simulink model "untitled_restored_from_autosave"  (R2021b)
settings: Solver=VariableStepAuto  StartTime=0.0  StopTime=100  RelTol=1e-3
libraries: uavalgslib x2, robotcorelib x1, simulink_extras x1, uavutilslib x1
settings Model: Creator=Jihoon Lee  LastModifiedBy=Jihoon Lee

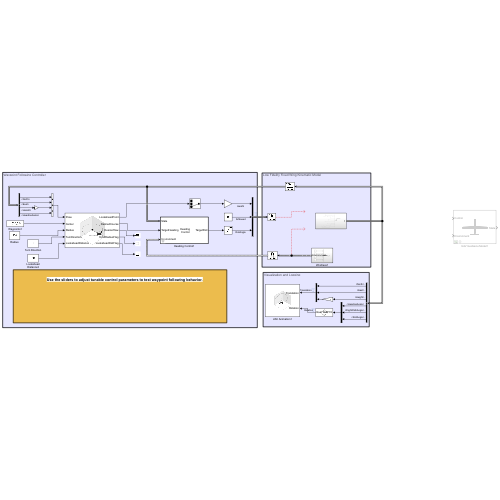
[thumbnail: Simulink's stored preview of the top-level diagram]
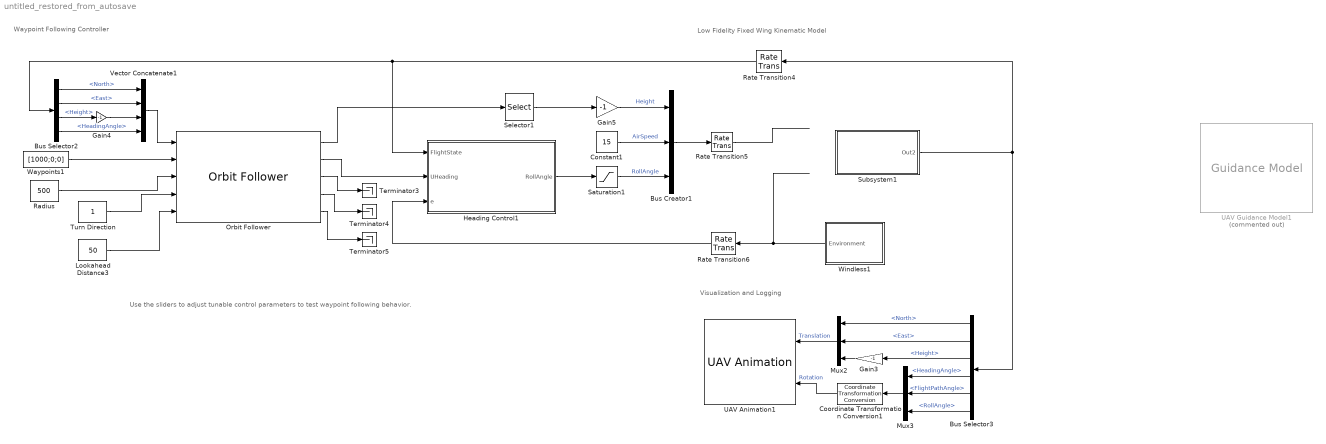
== system untitled_restored_from_autosave ==
  note: Waypoint Following Controller
  note: Use the sliders to adjust tunable control parameters to test waypoint following behavior.
  note: Low Fidelity Fixed Wing Kinematic Model
  note: Visualization and Logging
  Bus Creator1 : BusCreator  Inputs=3  OutDataTypeStr=Bus: FixedWingControlBus  NonVirtualBus=on
  Bus Selector2 : BusSelector  OutputSignals=North,East,Height,HeadingAngle
  Bus Selector3 : BusSelector  OutputSignals=North,East,Height,HeadingAngle,FlightPathAngle,RollAngle
  Constant1 : Constant  Value=15
  Coordinate Transformation Conversion1 : robotcorelib/Coordinate Transformation Conversion  InputRepresentation=Euler Angles  InputEulerSequence=ZYX  ShowTrVecInputPort=on  OutputRepresentation=Quaternion  OutputEulerSequence=ZYX  ShowTrVecOutputPort=on  SimulateUsing=Code generation
      settings: SourceProductBaseCode=NV,RO,RR,UV
  Gain3 : Gain  Gain=-1
  Gain4 : Gain  Gain=-1
  Gain5 : Gain  Gain=-1
  Heading Control1 : MATLAB Function  TreatAsAtomicUnit=on  mask(Fixed Wing Heading Controller){PHeadingAngle=0.39}
      mask prompts: PHeadingAngle "Heading Control Gain"
      mask help: P controller that regulates fixed wing UAV heading direction through controlling its roll angle. This controller requires that the plane is flying under coordinated flight condition.
  Lookahead Distance3 : Constant  Value=50
  Mux2 : Mux  Inputs=3
  Mux3 : Mux  Inputs=3
  Orbit Follower : uavalgslib/Orbit Follower  UAVType=fixed-wing  MinOrbitRadius=1  MinLookaheadDistance=0.1  ExternalReset=none  ShowCrossTrackErrorOutput=off  ShowNumTurnsOutput=off  SimulateUsing=Interpreted execution
      settings: SourceProductBaseCode=UV
  Radius : Constant  Value=500
  Rate Transition4 : RateTransition  OutPortSampleTime=0.01
  Rate Transition5 : RateTransition  OutPortSampleTime=0.1
  Rate Transition6 : RateTransition  OutPortSampleTime=0.01
  Saturation1 : Saturate  UpperLimit=20/180*pi  LowerLimit=-20/180*pi
  Selector1 : Selector  InputPortWidth=3  IndexOptions=Index vector (dialog)  Indices=[3]  OutputSizes=1
  Subsystem1 : Subsystem
  Terminator3 : Terminator
  Terminator4 : Terminator
  Terminator5 : Terminator
  Turn Direction : Constant
  UAV Animation1 : uavutilslib/UAV Animation  UAVType=FixedWing  UAVSize=50  InertialZDirection=Down  SampleTime=0.1
      settings: SourceProductBaseCode=UV
  UAV Guidance Model1 : uavalgslib/Guidance Model  Commented=on  ModelType=FixedWingGuidance  SpecifiedDataType=double  SimulateUsing=Code generation  InitialWorldPositionMultirotor=[0; 0; 0]  InitialWorldVelocityMultirotor=[0; 0; 0]  InitialEulerZYXMultirotor=[0; 0; 0]  InitialBodyAngularRateRPYMultirotor=[0; 0; 0]  InitialThrustMultirotor=0  InitialNorthFixedWing=0  InitialEastFixedWing=0  InitialHeightFixedWing=0  InitialAirSpeedFixedWing=15  InitialHeadingAngleFixedWing=0  InitialFlightPathAngleFixedWing=0  InitialRollAngleFixedWing=0  InitialRollAngleRateFixedWing=0  PDRollMultirotor=[3402.97,116.67]  PDPitchMultirotor=[3402.97, 116.67]  PYawRateMultirotor=1950  PThrustMultirotor=3900  MassMultirotor=0.1  PHeightFixedWing=3.9  PHeadingAngleFixedWing=3.9  PFlightPathAngleFixedWing=39  PDRollFixedWing=[5.9414, 3.9]  PAirSpeedFixedWing=1  FlightPathAngleLimitsFixedWing=[-pi/6, pi/6]  StateBusName='FixedWingStateBus'  ControlBusName='FixedWingControlBus'  EnvironmentBusName='FixedWingEnvironmentBus'  DataType=double
      settings: SourceProductBaseCode=UV
  Vector Concatenate1 : Concatenate  NumInputs=4
  Waypoints1 : Constant  Value=[1000;0;0]  VectorParams1D=off
  Windless1 : Subsystem  VariantControl=NoWind
  wires:
  Bus Selector3/4 -> Mux3/1  "<HeadingAngle>"
  Orbit Follower/4 -> Terminator4/1
  Saturation1/1 -> Bus Creator1/3  "RollAngle"
  Bus Selector3/3 -> Gain3/1  "<Height>"
  Bus Creator1/1 -> Rate Transition5/1
  Rate Transition4/1 -> Heading Control1/1(FlightState), Bus Selector2/1
  Subsystem1/1(Out2) -> Bus Selector3/1, Rate Transition4/1
  Bus Selector2/1 -> Vector Concatenate1/1  "<North>"
  Bus Selector3/6 -> Mux3/3  "<RollAngle>"
  Orbit Follower/3 -> Terminator3/1
  Gain5/1 -> Bus Creator1/1  "Height"
  Radius/1 -> Orbit Follower/3
  Rate Transition5/1 -> ?
  Bus Selector3/1 -> Mux2/1  "<North>"
  Orbit Follower/5 -> Terminator5/1
  Selector1/1 -> Gain5/1
  Gain4/1 -> Vector Concatenate1/3
  Orbit Follower/1 -> Selector1/1
  Heading Control1/1(RollAngle) -> Saturation1/1
  Gain3/1 -> Mux2/3
  Constant1/1 -> Bus Creator1/2  "AirSpeed"
  Bus Selector3/5 -> Mux3/2  "<FlightPathAngle>"
  Coordinate Transformation Conversion1/1 -> UAV Animation1/2  "Rotation"
  Windless1/1(Environment) -> Rate Transition6/1
  Bus Selector2/2 -> Vector Concatenate1/2  "<East>"
  Bus Selector2/4 -> Vector Concatenate1/4  "<HeadingAngle>"
  Mux2/1 -> UAV Animation1/1  "Translation"
  Mux3/1 -> Coordinate Transformation Conversion1/1
  Bus Selector3/2 -> Mux2/2  "<East>"
  Waypoints1/1 -> Orbit Follower/2
  Vector Concatenate1/1 -> Orbit Follower/1
  Orbit Follower/2 -> Heading Control1/2(UHeading)
  Turn Direction/1 -> Orbit Follower/4
  Rate Transition6/1 -> Heading Control1/3(e)
  Lookahead Distance3/1 -> Orbit Follower/5
  Bus Selector2/3 -> Gain4/1  "<Height>"

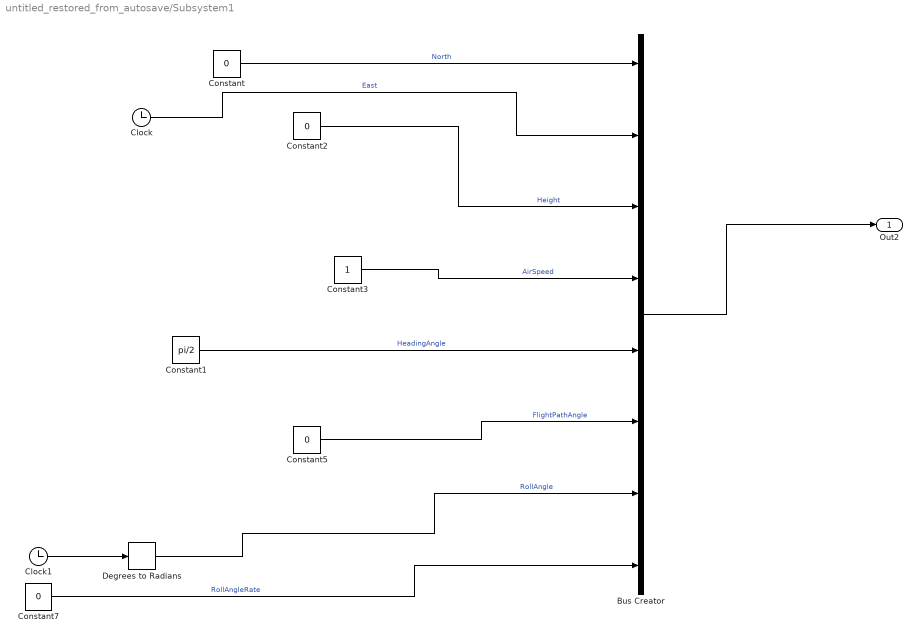
== system untitled_restored_from_autosave/Subsystem1 ==
  Bus Creator : BusCreator  Inputs=8
  Clock : Clock
  Clock1 : Clock
  Constant{,2,5,7} (4 alike) : Constant  Value=0
  Constant1 : Constant  Value=pi/2
  Constant3 : Constant
  Degrees to Radians : simulink_extras/Transformations/Degrees to Radians
  Out2 : Outport
  wires:
  Constant1/1 -> Bus Creator/5  "HeadingAngle"
  Constant2/1 -> Bus Creator/3  "Height"
  Clock/1 -> Bus Creator/2  "East"
  Constant/1 -> Bus Creator/1  "North"
  Constant5/1 -> Bus Creator/6  "FlightPathAngle"
  Clock1/1 -> Degrees to Radians/1
  Constant7/1 -> Bus Creator/8  "RollAngleRate"
  Constant3/1 -> Bus Creator/4  "AirSpeed"
  Bus Creator/1 -> Out2/1
  Degrees to Radians/1 -> Bus Creator/7  "RollAngle"

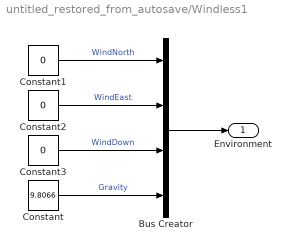
== system untitled_restored_from_autosave/Windless1 ==
  Bus Creator : BusCreator  Inputs=4  OutDataTypeStr=Bus: FixedWingEnvironmentBus  NonVirtualBus=on
  Constant : Constant  Value=9.8066
  Constant1 : Constant  Value=0
  Constant2 : Constant  Value=0
  Constant3 : Constant  Value=0
  Environment : Outport  VectorParamsAs1DForOutWhenUnconnected=off
  wires:
  Constant2/1 -> Bus Creator/2  "WindEast"
  Constant3/1 -> Bus Creator/3  "WindDown"
  Constant1/1 -> Bus Creator/1  "WindNorth"
  Bus Creator/1 -> Environment/1
  Constant/1 -> Bus Creator/4  "Gravity"

== matlab function untitled_restored_from_autosave/Heading Control1 ==
  data: FlightState input Bus: FixedWingStateBus; UHeading input; RollAngle output size=[1 1]; e input Bus: FixedWingEnvironmentBus; PHeadingAngle parameter
function RollAngle = fcn(FlightState, UHeading, e, PHeadingAngle)
    
    Va = FlightState.AirSpeed;
    HeadingAngle = FlightState.HeadingAngle;
    FlightPathAngle = FlightState.FlightPathAngle;
    
    YawAngle = HeadingAngle - asin((1/Va)*[e.WindNorth, e.WindEast]*[-sin(HeadingAngle); cos(HeadingAngle)]);
    b = [cos(HeadingAngle)*cos(FlightPathAngle), sin(HeadingAngle)*cos(FlightPathAngle), -sin(FlightPathAngle)]*[e.WindNorth; e.WindEast; e.WindDown];
    c = [e.WindNorth, e.WindEast, e.WindDown]*[e.WindNorth; e.WindEast; e.WindDown]- Va^2;
    Vg = -b+sqrt(b^2-c);
    
    RollAngle = atan2(PHeadingAngle*angdiff(HeadingAngle,UHeading)*Vg,e.Gravity*cos(HeadingAngle-YawAngle));
